simulink model "ElectricVehicleThermalManagementWithHeatPump_2026a_version"  (R2026a)
settings: Solver=VariableStepAuto  StopTime=3600  AbsTol=1e-3
PreLoadFcn:
  | init_nmpc
InitFcn:
  | init_nmpc
model workspace: external: MATLAB File ElectricVehicleThermalManagementWithHeatPumpParameters.m (data not in the file)
values from neighbouring files (symbols this model uses):
  battery_C1_LUT = [1913.6 12447 30609 ... (first row only)    [ElectricVehicleThermalManagementWithHeatPumpParameters.m]
  battery_capacity_LUT = [280.081 276.25 276.392]    [ElectricVehicleThermalManagementWithHeatPumpParameters.m]
  battery_cell_cp = 795    [ElectricVehicleThermalManagementWithHeatPumpParameters.m]
  battery_cell_mass = 2.5    [ElectricVehicleThermalManagementWithHeatPumpParameters.m]
  battery_Em_LUT = [3.4966 3.5057 3.5148 ... (first row only)    [ElectricVehicleThermalManagementWithHeatPumpParameters.m]
  battery_N_cells = 20    [ElectricVehicleThermalManagementWithHeatPumpParameters.m]
  battery_Qe_init = 0    [ElectricVehicleThermalManagementWithHeatPumpParameters.m]
  battery_R0_LUT = [0.0117 0.0085 0.009 ... (first row only)    [ElectricVehicleThermalManagementWithHeatPumpParameters.m]
  battery_R1_LUT = [0.0109 0.0029 0.0013 ... (first row only)    [ElectricVehicleThermalManagementWithHeatPumpParameters.m]
  battery_SOC_LUT = [0; 0.1; 0.25; 0.5; 0.75; 0.9; 1]    [ElectricVehicleThermalManagementWithHeatPumpParameters.m]
  battery_T_init = -5    [ElectricVehicleThermalManagementWithHeatPumpParameters.m]
  battery_temperature_LUT = [5 20 40]    [ElectricVehicleThermalManagementWithHeatPumpParameters.m]
  cabin_duct_area = 0.04    [ElectricVehicleThermalManagementWithHeatPumpParameters.m]
  cabin_T_init = -5    [ElectricVehicleThermalManagementWithHeatPumpParameters.m]
  chiller_area_primary = 0.43982297150257105    (= 0.439822971503)    [ElectricVehicleThermalManagementWithHeatPumpParameters.m]
  chiller_N_baffles = 3    [ElectricVehicleThermalManagementWithHeatPumpParameters.m]
  chiller_N_tubes = 100    [ElectricVehicleThermalManagementWithHeatPumpParameters.m]
  chiller_tube_D = 0.0035    [ElectricVehicleThermalManagementWithHeatPumpParameters.m]
  chiller_tube_L = 0.4    [ElectricVehicleThermalManagementWithHeatPumpParameters.m]
  chiller_wall_conductivity = 240    [ElectricVehicleThermalManagementWithHeatPumpParameters.m]
  chiller_wall_thickness = 0.0001    [ElectricVehicleThermalManagementWithHeatPumpParameters.m]
  cond_evap_air_area_flow = 0.3906    [ElectricVehicleThermalManagementWithHeatPumpParameters.m]
  cond_evap_air_area_primary = 1.4834999999999998    (= 1.4835)    [ElectricVehicleThermalManagementWithHeatPumpParameters.m]
  cond_evap_W = 0.015    [ElectricVehicleThermalManagementWithHeatPumpParameters.m]
  cond_evap_wall_conductivity = 240    [ElectricVehicleThermalManagementWithHeatPumpParameters.m]
  cond_evap_wall_thickness = 0.0001    [ElectricVehicleThermalManagementWithHeatPumpParameters.m]
  coolant_channel_D = 0.0092    [ElectricVehicleThermalManagementWithHeatPumpParameters.m]
  coolant_pipe_D = 0.019    [ElectricVehicleThermalManagementWithHeatPumpParameters.m]
  coolant_T_init = -5    [ElectricVehicleThermalManagementWithHeatPumpParameters.m]
  coolant_tank_area = 0.0121    [ElectricVehicleThermalManagementWithHeatPumpParameters.m]
  coolant_tank_volume = 1.25    [ElectricVehicleThermalManagementWithHeatPumpParameters.m]
  coolant_valve_D_ratio_max = 0.95    [ElectricVehicleThermalManagementWithHeatPumpParameters.m]
  coolant_valve_D_ratio_min = 0.001    [ElectricVehicleThermalManagementWithHeatPumpParameters.m]
  coolant_valve_displacement = 0.0063    [ElectricVehicleThermalManagementWithHeatPumpParameters.m]
  coolant_valve_S_max = 0.0053    [ElectricVehicleThermalManagementWithHeatPumpParameters.m]
  evaporator_air_area_flow = 0.12    [ElectricVehicleThermalManagementWithHeatPumpParameters.m]
  evaporator_air_area_primary = 0.4323    [ElectricVehicleThermalManagementWithHeatPumpParameters.m]
  evaporator_W = 0.015    [ElectricVehicleThermalManagementWithHeatPumpParameters.m]
  evaporator_wall_conductivity = 240    [ElectricVehicleThermalManagementWithHeatPumpParameters.m]
  evaporator_wall_thickness = 0.0001    [ElectricVehicleThermalManagementWithHeatPumpParameters.m]
  expansion_valve_D_ratio_max = 0.9    [ElectricVehicleThermalManagementWithHeatPumpParameters.m]
  hex_area_primary = 0.070371675440411369    (= 0.0703716754404)    [ElectricVehicleThermalManagementWithHeatPumpParameters.m]
  hex_N_tubes = 64    [ElectricVehicleThermalManagementWithHeatPumpParameters.m]
  hex_tube_D = 0.0035    [ElectricVehicleThermalManagementWithHeatPumpParameters.m]
  hex_wall_conductivity = 240    [ElectricVehicleThermalManagementWithHeatPumpParameters.m]
  hex_wall_thickness = 0.0001    [ElectricVehicleThermalManagementWithHeatPumpParameters.m]
  inner_cond_air_area_flow = 0.1953    [ElectricVehicleThermalManagementWithHeatPumpParameters.m]
  inner_cond_air_area_primary = 0.99520000000000008    (= 0.9952)    [ElectricVehicleThermalManagementWithHeatPumpParameters.m]
  inner_cond_W = 0.02    [ElectricVehicleThermalManagementWithHeatPumpParameters.m]
  inner_cond_wall_conductivity = 240    [ElectricVehicleThermalManagementWithHeatPumpParameters.m]
  inner_cond_wall_thickness = 0.0001    [ElectricVehicleThermalManagementWithHeatPumpParameters.m]
  pump_speed_max = 1000    [ElectricVehicleThermalManagementWithHeatPumpParameters.m]
  radiator_air_area_flow = 0.097499999999999989    (= 0.0975)    [ElectricVehicleThermalManagementWithHeatPumpParameters.m]
  radiator_air_area_primary = 0.43687499999999996    (= 0.436875)    [ElectricVehicleThermalManagementWithHeatPumpParameters.m]
  radiator_W = 0.015    [ElectricVehicleThermalManagementWithHeatPumpParameters.m]
  radiator_wall_conductivity = 240    [ElectricVehicleThermalManagementWithHeatPumpParameters.m]
  radiator_wall_thickness = 0.0001    [ElectricVehicleThermalManagementWithHeatPumpParameters.m]
  refrigerant_p_init = 0.25    [ElectricVehicleThermalManagementWithHeatPumpParameters.m]
  refrigerant_pipe_D = 0.01    [ElectricVehicleThermalManagementWithHeatPumpParameters.m]
  refrigerant_valve_D_ratio_max = 0.95    [ElectricVehicleThermalManagementWithHeatPumpParameters.m]
  refrigerant_valve_displacement = 0.005    [ElectricVehicleThermalManagementWithHeatPumpParameters.m]
libraries: fl_lib x227, nesl_utility x162, SimscapeFluids_lib x30, LiBatteryElements_lib x16, slpidlib x3, SignalEditorBlockLib x1
(part 11 of 13)

== system ElectricVehicleThermalManagementWithHeatPump_2026a_version/Controls/T_battery ==
  MinMax : MinMax  Function=max  Inputs=4
  T_battery : Outport
  wires:
  MinMax/1 -> T_battery/1
  [T_battery1] -> MinMax/1
  [T_battery4] -> MinMax/4
  [T_battery2] -> MinMax/2
  [T_battery3] -> MinMax/3

== system ElectricVehicleThermalManagementWithHeatPump_2026a_version/Controls/Thermal Mode ==
  note: 0 = Off
      |
      | 1 = Cold loop
      |
      | 2 = Heat pump
  T_env : Inport
  rpm_comp : Inport  Port=2
  Mode Selection : Subsystem
  Mode Transition : Subsystem
  Scope : Scope
      settings: ActiveDisplayYMinimum=0.9  ActiveDisplayYMaximum=1.1
  To Workspace : ToWorkspace  VariableName=thermal_mode  SampleTime=-1
  thermal_mode : Outport
  wires:
  T_env/1 -> Mode Selection/1(T_env)
  Mode Selection/1(setpoint) -> Scope/1, Mode Transition/1(setpoint)
  Mode Transition/1(thermal_mode) -> To Workspace/1, thermal_mode/1
  rpm_comp/1 -> Mode Transition/2(rpm_comp)

== system ElectricVehicleThermalManagementWithHeatPump_2026a_version/Controls/Valves Control ==
  thermal_mode : Inport
  T_coolant_inverter_out : Inport  Port=2
  T_coolant_battery_in : Inport  Port=3
  T_env : Inport  Port=4
  Chiller Expansion Valve : Subsystem
  Evaporator Expansion Valve : Subsystem
  Heat Pump Expansion Valve : Subsystem
  Radiator 3-Way Valve : Subsystem
  Refrigerant and Air 3-Way Valve : Subsystem
  To Workspace1 : ToWorkspace  VariableName=clntInverterTemp_out  SampleTime=-1
  To Workspace2 : ToWorkspace  VariableName=clntBatTemp_in  SampleTime=-1
  To Workspace3 : ToWorkspace  VariableName=envTemp  SampleTime=-1
  To Workspace4 : ToWorkspace  VariableName=cmdRefByPass  SampleTime=-1
  To Workspace5 : ToWorkspace  VariableName=cmdBlendAir  SampleTime=-1
  To Workspace6 : ToWorkspace  VariableName=cmdRadByPass  SampleTime=-1
  To Workspace7 : ToWorkspace  VariableName=cmdExvChill  SampleTime=-1
  To Workspace8 : ToWorkspace  VariableName=cmdExvEvap  SampleTime=-1
  To Workspace9 : ToWorkspace  VariableName=cmdExvHeatpump  SampleTime=-1
  cmd_refrig_bypass : Outport
  cmd_blend_air : Outport  Port=2
  cmd_rad_bypass : Outport  Port=3
  cmd_exv_chiller : Outport  Port=4
  cmd_exv_evap : Outport  Port=5
  cmd_exv_heatpump : Outport  Port=6
  wires:
  Refrigerant and Air 3-Way Valve/1(cmd_refrig_bypass) -> To Workspace4/1, cmd_refrig_bypass/1
  Refrigerant and Air 3-Way Valve/2(cmd_blend_air) -> To Workspace5/1, cmd_blend_air/1
  T_env/1 -> To Workspace3/1, Heat Pump Expansion Valve/2(T_env), Evaporator Expansion Valve/2(T_env)
  T_coolant_battery_in/1 -> To Workspace2/1, Chiller Expansion Valve/2(T_coolant_battery_in)
  T_coolant_inverter_out/1 -> To Workspace1/1, Radiator 3-Way Valve/2(T_coolant_inverter_out)
  thermal_mode/1 -> Radiator 3-Way Valve/1(thermal_mode), Chiller Expansion Valve/1(thermal_mode), Evaporator Expansion Valve/1(thermal_mode), Heat Pump Expansion Valve/1(thermal_mode), Refrigerant and Air 3-Way Valve/1(thermal_mode)
  Radiator 3-Way Valve/1(cmd_rad_bypass) -> To Workspace6/1, cmd_rad_bypass/1
  Chiller Expansion Valve/1(cmd_exv_chiller) -> To Workspace7/1, cmd_exv_chiller/1
  Evaporator Expansion Valve/1(cmd_exv_evap) -> To Workspace8/1, cmd_exv_evap/1
  Heat Pump Expansion Valve/1(cmd_exv_heatpump) -> To Workspace9/1, cmd_exv_heatpump/1

== system ElectricVehicleThermalManagementWithHeatPump_2026a_version/Evaporator/SR7 ==
  Flow Rate Sensor (2P) : fl_lib/Two-Phase Fluid/Sensors/Flow Rate Sensor (2P)  mass_flow_measure=true  volumetric_flow_measure=false  energy_flow_measure=true
  PS-Simulink Converter : nesl_utility/PS-Simulink Converter  PhysicalDomain=network_engine_domain  SubClassName=ps_output  LeftPortType=input  RightPortType=output  PseudoPeriodic=off  Frequencies=[]  VectorFormat=inherit  Unit=W  AffineConversion=off
  PS-Simulink Converter{1..4} (4 alike) : nesl_utility/PS-Simulink Converter  PhysicalDomain=network_engine_domain  SubClassName=ps_output  LeftPortType=input  RightPortType=output  PseudoPeriodic=off  Frequencies=[]  VectorFormat=inherit  Unit=inherit  AffineConversion=off
  "Pressure, Temperature & Internal Energy Sensor (2P)" : fl_lib/Two-Phase Fluid/Sensors/Pressure, Temperature & Internal Energy Sensor (2P)  reference=foundation.enum.MeasurementReference.absolute  pressure=true  pressure_spec=foundation.enum.PressureMeasementSpec.Absolute  temperature=false  internal_energy=false
  Thermodynamic Properties Sensor (2P) : fl_lib/Two-Phase Fluid/Sensors/Thermodynamic Properties Sensor (2P)  temperature=true  enthalpy=true  density=true  specific_volume=false  entropy=true
  To Workspace : ToWorkspace  VariableName=refEvapTemp_in  SampleTime=-1
  To Workspace1 : ToWorkspace  VariableName=refEvapH_in  SampleTime=-1
  To Workspace2 : ToWorkspace  VariableName=refEvapRho_in  SampleTime=-1
  To Workspace3 : ToWorkspace  VariableName=refEvapPres_in  SampleTime=-1
  A : PMIOPort  Side=Left
  B : PMIOPort  Port=2  Side=Right
  tag scope: Phi_evap_in=global
  wires:
  PS-Simulink Converter/1 -> [Phi_evap_in]
  PS-Simulink Converter1/1 -> To Workspace/1
  PS-Simulink Converter2/1 -> To Workspace1/1
  PS-Simulink Converter3/1 -> To Workspace2/1
  PS-Simulink Converter4/1 -> To Workspace3/1
  connections:
  PS-Simulink Converter/LConn1 -- Flow Rate Sensor (2P)/RConn3
  B/RConn1 -- Flow Rate Sensor (2P)/RConn1
  Thermodynamic Properties Sensor (2P)/LConn1 -- A/RConn1 -- "Pressure, Temperature & Internal Energy Sensor (2P)"/LConn1 -- Flow Rate Sensor (2P)/LConn1
  PS-Simulink Converter1/LConn1 -- Thermodynamic Properties Sensor (2P)/RConn1
  PS-Simulink Converter2/LConn1 -- Thermodynamic Properties Sensor (2P)/RConn2
  PS-Simulink Converter3/LConn1 -- Thermodynamic Properties Sensor (2P)/RConn3
  PS-Simulink Converter4/LConn1 -- "Pressure, Temperature & Internal Energy Sensor (2P)"/RConn1

== system ElectricVehicleThermalManagementWithHeatPump_2026a_version/Evaporator/SR8 ==
  Flow Rate Sensor (2P) : fl_lib/Two-Phase Fluid/Sensors/Flow Rate Sensor (2P)  mass_flow_measure=true  volumetric_flow_measure=false  energy_flow_measure=true
  PS-Simulink Converter : nesl_utility/PS-Simulink Converter  PhysicalDomain=network_engine_domain  SubClassName=ps_output  LeftPortType=input  RightPortType=output  PseudoPeriodic=off  Frequencies=[]  VectorFormat=inherit  Unit=W  AffineConversion=off
  PS-Simulink Converter1 : nesl_utility/PS-Simulink Converter  PhysicalDomain=network_engine_domain  SubClassName=ps_output  LeftPortType=input  RightPortType=output  PseudoPeriodic=off  Frequencies=[]  VectorFormat=inherit  Unit=MPa  AffineConversion=off
  PS-Simulink Converter2 : nesl_utility/PS-Simulink Converter  PhysicalDomain=network_engine_domain  SubClassName=ps_output  LeftPortType=input  RightPortType=output  PseudoPeriodic=off  Frequencies=[]  VectorFormat=inherit  Unit=inherit  AffineConversion=off
  PS-Simulink Converter3 : nesl_utility/PS-Simulink Converter  PhysicalDomain=network_engine_domain  SubClassName=ps_output  LeftPortType=input  RightPortType=output  PseudoPeriodic=off  Frequencies=[]  VectorFormat=inherit  Unit=inherit  AffineConversion=off
  PS-Simulink Converter4 : nesl_utility/PS-Simulink Converter  PhysicalDomain=network_engine_domain  SubClassName=ps_output  LeftPortType=input  RightPortType=output  PseudoPeriodic=off  Frequencies=[]  VectorFormat=inherit  Unit=inherit  AffineConversion=off
  "Pressure, Temperature & Internal Energy Sensor (2P)" : fl_lib/Two-Phase Fluid/Sensors/Pressure, Temperature & Internal Energy Sensor (2P)  reference=foundation.enum.MeasurementReference.absolute  pressure=true  pressure_spec=foundation.enum.PressureMeasementSpec.Absolute  temperature=false  internal_energy=false
  Thermodynamic Properties Sensor (2P) : fl_lib/Two-Phase Fluid/Sensors/Thermodynamic Properties Sensor (2P)  temperature=true  enthalpy=true  density=true  specific_volume=false  entropy=true
  To Workspace : ToWorkspace  VariableName=refEvapPress_out  SampleTime=-1
  To Workspace1 : ToWorkspace  VariableName=refEvapTemp_out  SampleTime=-1
  To Workspace2 : ToWorkspace  VariableName=refEvapH_out  SampleTime=-1
  To Workspace3 : ToWorkspace  VariableName=refEvapRho_out  SampleTime=-1
  A : PMIOPort  Side=Left
  B : PMIOPort  Port=2  Side=Right
  tag scope: Phi_evap_out=global, p_evap_out=global
  wires:
  PS-Simulink Converter/1 -> [Phi_evap_out]
  PS-Simulink Converter1/1 -> To Workspace/1, [p_evap_out]
  PS-Simulink Converter2/1 -> To Workspace1/1
  PS-Simulink Converter3/1 -> To Workspace2/1
  PS-Simulink Converter4/1 -> To Workspace3/1
  connections:
  PS-Simulink Converter/LConn1 -- Flow Rate Sensor (2P)/RConn3
  B/RConn1 -- Flow Rate Sensor (2P)/RConn1
  Thermodynamic Properties Sensor (2P)/LConn1 -- A/RConn1 -- "Pressure, Temperature & Internal Energy Sensor (2P)"/LConn1 -- Flow Rate Sensor (2P)/LConn1
  PS-Simulink Converter1/LConn1 -- "Pressure, Temperature & Internal Energy Sensor (2P)"/RConn1
  PS-Simulink Converter2/LConn1 -- Thermodynamic Properties Sensor (2P)/RConn1
  PS-Simulink Converter3/LConn1 -- Thermodynamic Properties Sensor (2P)/RConn2
  PS-Simulink Converter4/LConn1 -- Thermodynamic Properties Sensor (2P)/RConn3

== system ElectricVehicleThermalManagementWithHeatPump_2026a_version/Heat Exchanger/SR5 ==
  Flow Rate Sensor (2P) : fl_lib/Two-Phase Fluid/Sensors/Flow Rate Sensor (2P)  mass_flow_measure=true  volumetric_flow_measure=false  energy_flow_measure=true
  PS-Simulink Converter : nesl_utility/PS-Simulink Converter  PhysicalDomain=network_engine_domain  SubClassName=ps_output  LeftPortType=input  RightPortType=output  PseudoPeriodic=off  Frequencies=[]  VectorFormat=inherit  Unit=W  AffineConversion=off
  PS-Simulink Converter1 : nesl_utility/PS-Simulink Converter  PhysicalDomain=network_engine_domain  SubClassName=ps_output  LeftPortType=input  RightPortType=output  PseudoPeriodic=off  Frequencies=[]  VectorFormat=inherit  Unit=inherit  AffineConversion=off
  PS-Simulink Converter2 : nesl_utility/PS-Simulink Converter  PhysicalDomain=network_engine_domain  SubClassName=ps_output  LeftPortType=input  RightPortType=output  PseudoPeriodic=off  Frequencies=[]  VectorFormat=inherit  Unit=inherit  AffineConversion=off
  PS-Simulink Converter3 : nesl_utility/PS-Simulink Converter  PhysicalDomain=network_engine_domain  SubClassName=ps_output  LeftPortType=input  RightPortType=output  PseudoPeriodic=off  Frequencies=[]  VectorFormat=inherit  Unit=inherit  AffineConversion=off
  "Pressure, Temperature & Internal Energy Sensor (2P)" : fl_lib/Two-Phase Fluid/Sensors/Pressure, Temperature & Internal Energy Sensor (2P)  reference=foundation.enum.MeasurementReference.absolute  pressure=true  pressure_spec=foundation.enum.PressureMeasementSpec.Absolute  temperature=false  internal_energy=false
  Scope : Scope
      settings: DataLoggingVariableName=ScopeData4
  Scope1 : Scope
      settings: ActiveDisplayYMinimum=256.57304  ActiveDisplayYMaximum=268.20044  DataLoggingVariableName=ScopeData5
  Scope2 : Scope
      settings: DataLoggingVariableName=ScopeData6
  Thermodynamic Properties Sensor (2P) : fl_lib/Two-Phase Fluid/Sensors/Thermodynamic Properties Sensor (2P)  temperature=true  enthalpy=true  density=true  specific_volume=false  entropy=true
  To Workspace : ToWorkspace  VariableName=heatExchangerRefPress_inPa  SampleTime=-1
  To Workspace1 : ToWorkspace  VariableName=heatExchangerRefTemp_inK  SampleTime=-1
  To Workspace2 : ToWorkspace  VariableName=heatExchangerRefEnthaply_in  SampleTime=-1
  A : PMIOPort  Side=Left
  B : PMIOPort  Port=2  Side=Right
  tag scope: Phi_hex_in=global
  wires:
  PS-Simulink Converter/1 -> [Phi_hex_in]
  PS-Simulink Converter2/1 -> Scope/1, To Workspace/1
  PS-Simulink Converter1/1 -> Scope1/1, To Workspace1/1
  PS-Simulink Converter3/1 -> Scope2/1, To Workspace2/1
  connections:
  PS-Simulink Converter/LConn1 -- Flow Rate Sensor (2P)/RConn3
  B/RConn1 -- Flow Rate Sensor (2P)/RConn1
  Thermodynamic Properties Sensor (2P)/LConn1 -- A/RConn1 -- "Pressure, Temperature & Internal Energy Sensor (2P)"/LConn1 -- Flow Rate Sensor (2P)/LConn1
  PS-Simulink Converter1/LConn1 -- Thermodynamic Properties Sensor (2P)/RConn1
  PS-Simulink Converter2/LConn1 -- "Pressure, Temperature & Internal Energy Sensor (2P)"/RConn1
  Thermodynamic Properties Sensor (2P)/RConn2 -- PS-Simulink Converter3/LConn1

== system ElectricVehicleThermalManagementWithHeatPump_2026a_version/Heat Exchanger/SR6 ==
  Flow Rate Sensor (2P) : fl_lib/Two-Phase Fluid/Sensors/Flow Rate Sensor (2P)  mass_flow_measure=true  volumetric_flow_measure=false  energy_flow_measure=true
  PS-Simulink Converter : nesl_utility/PS-Simulink Converter  PhysicalDomain=network_engine_domain  SubClassName=ps_output  LeftPortType=input  RightPortType=output  PseudoPeriodic=off  Frequencies=[]  VectorFormat=inherit  Unit=W  AffineConversion=off
  PS-Simulink Converter1 : nesl_utility/PS-Simulink Converter  PhysicalDomain=network_engine_domain  SubClassName=ps_output  LeftPortType=input  RightPortType=output  PseudoPeriodic=off  Frequencies=[]  VectorFormat=inherit  Unit=inherit  AffineConversion=off
  PS-Simulink Converter2 : nesl_utility/PS-Simulink Converter  PhysicalDomain=network_engine_domain  SubClassName=ps_output  LeftPortType=input  RightPortType=output  PseudoPeriodic=off  Frequencies=[]  VectorFormat=inherit  Unit=inherit  AffineConversion=off
  PS-Simulink Converter3 : nesl_utility/PS-Simulink Converter  PhysicalDomain=network_engine_domain  SubClassName=ps_output  LeftPortType=input  RightPortType=output  PseudoPeriodic=off  Frequencies=[]  VectorFormat=inherit  Unit=inherit  AffineConversion=off
  "Pressure, Temperature & Internal Energy Sensor (2P)" : fl_lib/Two-Phase Fluid/Sensors/Pressure, Temperature & Internal Energy Sensor (2P)  reference=foundation.enum.MeasurementReference.absolute  pressure=true  pressure_spec=foundation.enum.PressureMeasementSpec.Absolute  temperature=false  internal_energy=false
  Scope : Scope
      settings: DataLoggingVariableName=ScopeData7
  Scope1 : Scope
      settings: ActiveDisplayYMinimum=256.25115  ActiveDisplayYMaximum=271.0073  DataLoggingVariableName=ScopeData8
  Scope2 : Scope
      settings: DataLoggingVariableName=ScopeData9
  Thermodynamic Properties Sensor (2P) : fl_lib/Two-Phase Fluid/Sensors/Thermodynamic Properties Sensor (2P)  temperature=true  enthalpy=true  density=true  specific_volume=false  entropy=true
  To Workspace : ToWorkspace  VariableName=heatExchangerRefPress_outPa  SampleTime=-1
  To Workspace1 : ToWorkspace  VariableName=heatExchangerRefTemp_outK  SampleTime=-1
  To Workspace2 : ToWorkspace  VariableName=heatExchangerRefEnthaply_out  SampleTime=-1
  A : PMIOPort  Side=Left
  B : PMIOPort  Port=2  Side=Right
  tag scope: Phi_hex_out=global
  wires:
  PS-Simulink Converter/1 -> [Phi_hex_out]
  PS-Simulink Converter1/1 -> Scope/1, To Workspace/1
  PS-Simulink Converter2/1 -> Scope1/1, To Workspace1/1
  PS-Simulink Converter3/1 -> Scope2/1, To Workspace2/1
  connections:
  PS-Simulink Converter/LConn1 -- Flow Rate Sensor (2P)/RConn3
  B/RConn1 -- Flow Rate Sensor (2P)/RConn1
  Thermodynamic Properties Sensor (2P)/LConn1 -- A/RConn1 -- "Pressure, Temperature & Internal Energy Sensor (2P)"/LConn1 -- Flow Rate Sensor (2P)/LConn1
  PS-Simulink Converter1/LConn1 -- "Pressure, Temperature & Internal Energy Sensor (2P)"/RConn1
  PS-Simulink Converter2/LConn1 -- Thermodynamic Properties Sensor (2P)/RConn1
  PS-Simulink Converter3/LConn1 -- Thermodynamic Properties Sensor (2P)/RConn2

== system ElectricVehicleThermalManagementWithHeatPump_2026a_version/Inner Condenser/SR1 ==
  Flow Rate Sensor (2P) : fl_lib/Two-Phase Fluid/Sensors/Flow Rate Sensor (2P)  mass_flow_measure=true  volumetric_flow_measure=false  energy_flow_measure=true
  PS-Simulink Converter : nesl_utility/PS-Simulink Converter  PhysicalDomain=network_engine_domain  SubClassName=ps_output  LeftPortType=input  RightPortType=output  PseudoPeriodic=off  Frequencies=[]  VectorFormat=inherit  Unit=W  AffineConversion=off
  PS-Simulink Converter{1..4} (4 alike) : nesl_utility/PS-Simulink Converter  PhysicalDomain=network_engine_domain  SubClassName=ps_output  LeftPortType=input  RightPortType=output  PseudoPeriodic=off  Frequencies=[]  VectorFormat=inherit  Unit=inherit  AffineConversion=off
  "Pressure, Temperature & Internal Energy Sensor (2P)" : fl_lib/Two-Phase Fluid/Sensors/Pressure, Temperature & Internal Energy Sensor (2P)  reference=foundation.enum.MeasurementReference.absolute  pressure=true  pressure_spec=foundation.enum.PressureMeasementSpec.Absolute  temperature=false  internal_energy=false
  Scope{,1..3} (4 alike) : Scope
      Scope settings: DataLoggingVariableName=ScopeData13
      Scope1 settings: ActiveDisplayYMinimum=-0.00405  ActiveDisplayYMaximum=0.03648  DataLoggingVariableName=ScopeData14
      Scope2 settings: ActiveDisplayYMinimum=241.8446  ActiveDisplayYMaximum=454.07101  DataLoggingVariableName=ScopeData15
      Scope3 settings: DataLoggingVariableName=ScopeData16
  Thermodynamic Properties Sensor (2P) : fl_lib/Two-Phase Fluid/Sensors/Thermodynamic Properties Sensor (2P)  temperature=true  enthalpy=true  density=true  specific_volume=false  entropy=true
  To Workspace : ToWorkspace  VariableName=innerCondRefPress_inMPa  SampleTime=-1
  To Workspace1 : ToWorkspace  VariableName=RefMassFlowRate  SampleTime=-1
  To Workspace2 : ToWorkspace  VariableName=innerCondRefTemp_inK  SampleTime=-1
  To Workspace3 : ToWorkspace  VariableName=innerCondRefEnthaply_in  SampleTime=-1
  A : PMIOPort  Side=Left
  B : PMIOPort  Port=2  Side=Right
  tag scope: Phi_inner_cond_in=global
  wires:
  PS-Simulink Converter/1 -> [Phi_inner_cond_in]
  PS-Simulink Converter1/1 -> Scope/1, To Workspace/1
  PS-Simulink Converter2/1 -> Scope1/1, To Workspace1/1
  PS-Simulink Converter3/1 -> Scope2/1, To Workspace2/1
  PS-Simulink Converter4/1 -> Scope3/1, To Workspace3/1
  connections:
  PS-Simulink Converter/LConn1 -- Flow Rate Sensor (2P)/RConn3
  B/RConn1 -- Flow Rate Sensor (2P)/RConn1
  Thermodynamic Properties Sensor (2P)/LConn1 -- A/RConn1 -- "Pressure, Temperature & Internal Energy Sensor (2P)"/LConn1 -- Flow Rate Sensor (2P)/LConn1
  PS-Simulink Converter1/LConn1 -- "Pressure, Temperature & Internal Energy Sensor (2P)"/RConn1
  PS-Simulink Converter2/LConn1 -- Flow Rate Sensor (2P)/RConn2
  PS-Simulink Converter3/LConn1 -- Thermodynamic Properties Sensor (2P)/RConn1
  PS-Simulink Converter4/LConn1 -- Thermodynamic Properties Sensor (2P)/RConn2

== system ElectricVehicleThermalManagementWithHeatPump_2026a_version/Inner Condenser/SR2 ==
  Flow Rate Sensor (2P) : fl_lib/Two-Phase Fluid/Sensors/Flow Rate Sensor (2P)  mass_flow_measure=true  volumetric_flow_measure=false  energy_flow_measure=true
  PS-Simulink Converter : nesl_utility/PS-Simulink Converter  PhysicalDomain=network_engine_domain  SubClassName=ps_output  LeftPortType=input  RightPortType=output  PseudoPeriodic=off  Frequencies=[]  VectorFormat=inherit  Unit=W  AffineConversion=off
  PS-Simulink Converter1 : nesl_utility/PS-Simulink Converter  PhysicalDomain=network_engine_domain  SubClassName=ps_output  LeftPortType=input  RightPortType=output  PseudoPeriodic=off  Frequencies=[]  VectorFormat=inherit  Unit=MPa  AffineConversion=off
  PS-Simulink Converter2 : nesl_utility/PS-Simulink Converter  PhysicalDomain=network_engine_domain  SubClassName=ps_output  LeftPortType=input  RightPortType=output  PseudoPeriodic=off  Frequencies=[]  VectorFormat=inherit  Unit=inherit  AffineConversion=off
  PS-Simulink Converter3 : nesl_utility/PS-Simulink Converter  PhysicalDomain=network_engine_domain  SubClassName=ps_output  LeftPortType=input  RightPortType=output  PseudoPeriodic=off  Frequencies=[]  VectorFormat=inherit  Unit=inherit  AffineConversion=off
  "Pressure, Temperature & Internal Energy Sensor (2P)" : fl_lib/Two-Phase Fluid/Sensors/Pressure, Temperature & Internal Energy Sensor (2P)  reference=foundation.enum.MeasurementReference.absolute  pressure=true  pressure_spec=foundation.enum.PressureMeasementSpec.Absolute  temperature=false  internal_energy=false
  Thermodynamic Properties Sensor (2P) : fl_lib/Two-Phase Fluid/Sensors/Thermodynamic Properties Sensor (2P)  temperature=true  enthalpy=true  density=true  specific_volume=false  entropy=true
  To Workspace : ToWorkspace  VariableName=innerCondRefPress_outMpa  SampleTime=-1
  To Workspace1 : ToWorkspace  VariableName=innerCondRefTemp_outK  SampleTime=-1
  To Workspace2 : ToWorkspace  VariableName=innerCondRefEnthaply_out  SampleTime=-1
  A : PMIOPort  Side=Left
  B : PMIOPort  Port=2  Side=Right
  tag scope: Phi_inner_cond_out=global, p_inner_cond_out=global
  wires:
  PS-Simulink Converter/1 -> [Phi_inner_cond_out]
  PS-Simulink Converter1/1 -> To Workspace/1, [p_inner_cond_out]
  PS-Simulink Converter2/1 -> To Workspace1/1
  PS-Simulink Converter3/1 -> To Workspace2/1
  connections:
  PS-Simulink Converter/LConn1 -- Flow Rate Sensor (2P)/RConn3
  B/RConn1 -- Flow Rate Sensor (2P)/RConn1
  Thermodynamic Properties Sensor (2P)/LConn1 -- A/RConn1 -- "Pressure, Temperature & Internal Energy Sensor (2P)"/LConn1 -- Flow Rate Sensor (2P)/LConn1
  PS-Simulink Converter1/LConn1 -- "Pressure, Temperature & Internal Energy Sensor (2P)"/RConn1
  PS-Simulink Converter2/LConn1 -- Thermodynamic Properties Sensor (2P)/RConn1
  PS-Simulink Converter3/LConn1 -- Thermodynamic Properties Sensor (2P)/RConn2

== system ElectricVehicleThermalManagementWithHeatPump_2026a_version/Inverter/SC7 ==
  Flow Rate Sensor (TL) : fl_lib/Thermal Liquid/Sensors/Flow Rate Sensor (TL)  mass_flow_measure=true  volumetric_flow_measure=false  energy_flow_measure=true
  PS-Simulink Converter1 : nesl_utility/PS-Simulink Converter  PhysicalDomain=network_engine_domain  SubClassName=ps_output  LeftPortType=input  RightPortType=output  PseudoPeriodic=off  Frequencies=[]  VectorFormat=inherit  Unit=degC  AffineConversion=on
  Pressure & Temperature Sensor (TL) : fl_lib/Thermal Liquid/Sensors/Pressure & Temperature Sensor (TL)  reference=foundation.enum.MeasurementReference.absolute  pressure=true  pressure_spec=foundation.enum.PressureMeasementSpec.Absolute  temperature=true
  A : PMIOPort  Side=Left
  B : PMIOPort  Port=2  Side=Right
  tag scope: T_coolant_inverter_out=global
  wires:
  PS-Simulink Converter1/1 -> [T_coolant_inverter_out]
  connections:
  B/RConn1 -- Flow Rate Sensor (TL)/RConn1
  Flow Rate Sensor (TL)/LConn1 -- Pressure & Temperature Sensor (TL)/LConn1 -- A/RConn1
  PS-Simulink Converter1/LConn1 -- Pressure & Temperature Sensor (TL)/RConn2

== system ElectricVehicleThermalManagementWithHeatPump_2026a_version/Motor/SC5 ==
  Flow Rate Sensor (TL) : fl_lib/Thermal Liquid/Sensors/Flow Rate Sensor (TL)  mass_flow_measure=true  volumetric_flow_measure=false  energy_flow_measure=true
  PS-Simulink Converter : nesl_utility/PS-Simulink Converter  PhysicalDomain=network_engine_domain  SubClassName=ps_output  LeftPortType=input  RightPortType=output  PseudoPeriodic=off  Frequencies=[]  VectorFormat=inherit  Unit=W  AffineConversion=off
  Pressure & Temperature Sensor (TL) : fl_lib/Thermal Liquid/Sensors/Pressure & Temperature Sensor (TL)  reference=foundation.enum.MeasurementReference.absolute  pressure=true  pressure_spec=foundation.enum.PressureMeasementSpec.Absolute  temperature=true
  A : PMIOPort  Side=Left
  B : PMIOPort  Port=2  Side=Right
  tag scope: Phi_motor_in=global
  wires:
  PS-Simulink Converter/1 -> [Phi_motor_in]
  connections:
  B/RConn1 -- Flow Rate Sensor (TL)/RConn1
  Flow Rate Sensor (TL)/LConn1 -- Pressure & Temperature Sensor (TL)/LConn1 -- A/RConn1
  PS-Simulink Converter/LConn1 -- Flow Rate Sensor (TL)/RConn3

== system ElectricVehicleThermalManagementWithHeatPump_2026a_version/Motor/SC6 ==
  Flow Rate Sensor (TL) : fl_lib/Thermal Liquid/Sensors/Flow Rate Sensor (TL)  mass_flow_measure=true  volumetric_flow_measure=false  energy_flow_measure=true
  PS-Simulink Converter : nesl_utility/PS-Simulink Converter  PhysicalDomain=network_engine_domain  SubClassName=ps_output  LeftPortType=input  RightPortType=output  PseudoPeriodic=off  Frequencies=[]  VectorFormat=inherit  Unit=W  AffineConversion=off
  Pressure & Temperature Sensor (TL) : fl_lib/Thermal Liquid/Sensors/Pressure & Temperature Sensor (TL)  reference=foundation.enum.MeasurementReference.absolute  pressure=true  pressure_spec=foundation.enum.PressureMeasementSpec.Absolute  temperature=true
  A : PMIOPort  Side=Left
  B : PMIOPort  Port=2  Side=Right
  tag scope: Phi_motor_out=global
  wires:
  PS-Simulink Converter/1 -> [Phi_motor_out]
  connections:
  B/RConn1 -- Flow Rate Sensor (TL)/RConn1
  Flow Rate Sensor (TL)/LConn1 -- Pressure & Temperature Sensor (TL)/LConn1 -- A/RConn1
  PS-Simulink Converter/LConn1 -- Flow Rate Sensor (TL)/RConn3

== system ElectricVehicleThermalManagementWithHeatPump_2026a_version/Motor Pump/Heat Transfer ==
  Convective Heat Transfer : fl_lib/Thermal/Thermal Elements/Convective Heat Transfer  thermal_type=foundation.enum.constant_variable.constant  area=3 * coolant_tank_area m^2  heat_tr_coeff=20 W/(m^2 * K)  min_heat_tr_coeff=1e-3 W/(K*m^2)  T_specify=off  T_priority=None  T=0 K  T_nominal_specify=off  T_nominal_value=1  T_nominal_unit=K  Q_specify=off  Q_priority=None  Q=0 W  Q_nominal_specify=off  Q_nominal_value=1  Q_nominal_unit=W
  Convective Heat Transfer1 : fl_lib/Thermal/Thermal Elements/Convective Heat Transfer  thermal_type=foundation.enum.constant_variable.constant  area=3 * coolant_tank_area m^2  heat_tr_coeff=20 W/(m^2 * K)  min_heat_tr_coeff=1e-3 W/(K*m^2)  T_specify=off  T_priority=None  T=0 K  T_nominal_specify=off  T_nominal_value=1  T_nominal_unit=K  Q_specify=off  Q_priority=None  Q=0 W  Q_nominal_specify=off  Q_nominal_value=1  Q_nominal_unit=W
  Environment Temperature : fl_lib/Thermal/Thermal Sources/Controlled Temperature Source
  Simulink-PS Converter : nesl_utility/Simulink-PS Converter  PhysicalDomain=network_engine_domain  SubClassName=ps_input  LeftPortType=input  RightPortType=output  PseudoPeriodic=off  Frequencies=[]  NoiseDistribution=none  NoiseParameters=[]  Unit=degC  AffineConversion=on  FilteringAndDerivatives=provide  SimscapeFilterOrder=1  InputFilterTimeConstant=0.001  UdotUserProvided=0
  Thermal Reference : fl_lib/Thermal/Thermal Elements/Thermal Reference
  A : PMIOPort  Side=Right
  B : PMIOPort  Port=2  Side=Right
  wires:
  [T_env] -> Simulink-PS Converter/1
  connections:
  Simulink-PS Converter/RConn1 -- Environment Temperature/RConn1
  Thermal Reference/LConn1 -- Environment Temperature/RConn2
  Convective Heat Transfer/RConn1 -- Environment Temperature/LConn1 -- Convective Heat Transfer1/RConn1
  B/RConn1 -- Convective Heat Transfer1/LConn1
  A/RConn1 -- Convective Heat Transfer/LConn1

== system ElectricVehicleThermalManagementWithHeatPump_2026a_version/Radiator/SC1 ==
  Flow Rate Sensor (TL) : fl_lib/Thermal Liquid/Sensors/Flow Rate Sensor (TL)  mass_flow_measure=true  volumetric_flow_measure=false  energy_flow_measure=true
  PS-Simulink Converter : nesl_utility/PS-Simulink Converter  PhysicalDomain=network_engine_domain  SubClassName=ps_output  LeftPortType=input  RightPortType=output  PseudoPeriodic=off  Frequencies=[]  VectorFormat=inherit  Unit=W  AffineConversion=off
  PS-Simulink Converter1 : nesl_utility/PS-Simulink Converter  PhysicalDomain=network_engine_domain  SubClassName=ps_output  LeftPortType=input  RightPortType=output  PseudoPeriodic=off  Frequencies=[]  VectorFormat=inherit  Unit=inherit  AffineConversion=off
  Pressure & Temperature Sensor (TL) : fl_lib/Thermal Liquid/Sensors/Pressure & Temperature Sensor (TL)  reference=foundation.enum.MeasurementReference.absolute  pressure=true  pressure_spec=foundation.enum.PressureMeasementSpec.Absolute  temperature=true
  To Workspace : ToWorkspace  VariableName=clntRadTemp_in  SampleTime=-1
  A : PMIOPort  Side=Left
  B : PMIOPort  Port=2  Side=Right
  tag scope: Phi_rad_in=global
  wires:
  PS-Simulink Converter/1 -> [Phi_rad_in]
  PS-Simulink Converter1/1 -> To Workspace/1
  connections:
  PS-Simulink Converter/LConn1 -- Flow Rate Sensor (TL)/RConn3
  A/RConn1 -- Pressure & Temperature Sensor (TL)/LConn1 -- Flow Rate Sensor (TL)/LConn1
  B/RConn1 -- Flow Rate Sensor (TL)/RConn1
  PS-Simulink Converter1/LConn1 -- Pressure & Temperature Sensor (TL)/RConn2

== system ElectricVehicleThermalManagementWithHeatPump_2026a_version/Radiator/SC2 ==
  Flow Rate Sensor (TL) : fl_lib/Thermal Liquid/Sensors/Flow Rate Sensor (TL)  mass_flow_measure=true  volumetric_flow_measure=false  energy_flow_measure=true
  PS-Simulink Converter : nesl_utility/PS-Simulink Converter  PhysicalDomain=network_engine_domain  SubClassName=ps_output  LeftPortType=input  RightPortType=output  PseudoPeriodic=off  Frequencies=[]  VectorFormat=inherit  Unit=W  AffineConversion=off
  PS-Simulink Converter1 : nesl_utility/PS-Simulink Converter  PhysicalDomain=network_engine_domain  SubClassName=ps_output  LeftPortType=input  RightPortType=output  PseudoPeriodic=off  Frequencies=[]  VectorFormat=inherit  Unit=kg/s  AffineConversion=off
  PS-Simulink Converter2 : nesl_utility/PS-Simulink Converter  PhysicalDomain=network_engine_domain  SubClassName=ps_output  LeftPortType=input  RightPortType=output  PseudoPeriodic=off  Frequencies=[]  VectorFormat=inherit  Unit=inherit  AffineConversion=off
  Pressure & Temperature Sensor (TL) : fl_lib/Thermal Liquid/Sensors/Pressure & Temperature Sensor (TL)  reference=foundation.enum.MeasurementReference.absolute  pressure=true  pressure_spec=foundation.enum.PressureMeasementSpec.Absolute  temperature=true
  Scope : Scope
      settings: ActiveDisplayYMinimum=-0.01333  ActiveDisplayYMaximum=0.11994  DataLoggingVariableName=ScopeData4
  To Workspace : ToWorkspace  VariableName=clntRadTemp_out  SampleTime=-1
  A : PMIOPort  Side=Left
  B : PMIOPort  Port=2  Side=Right
  tag scope: Phi_rad_out=global
  wires:
  PS-Simulink Converter/1 -> [Phi_rad_out]
  PS-Simulink Converter1/1 -> Scope/1
  PS-Simulink Converter2/1 -> To Workspace/1
  connections:
  PS-Simulink Converter/LConn1 -- Flow Rate Sensor (TL)/RConn3
  A/RConn1 -- Pressure & Temperature Sensor (TL)/LConn1 -- Flow Rate Sensor (TL)/LConn1
  B/RConn1 -- Flow Rate Sensor (TL)/RConn1
  PS-Simulink Converter1/LConn1 -- Flow Rate Sensor (TL)/RConn2
  PS-Simulink Converter2/LConn1 -- Pressure & Temperature Sensor (TL)/RConn2

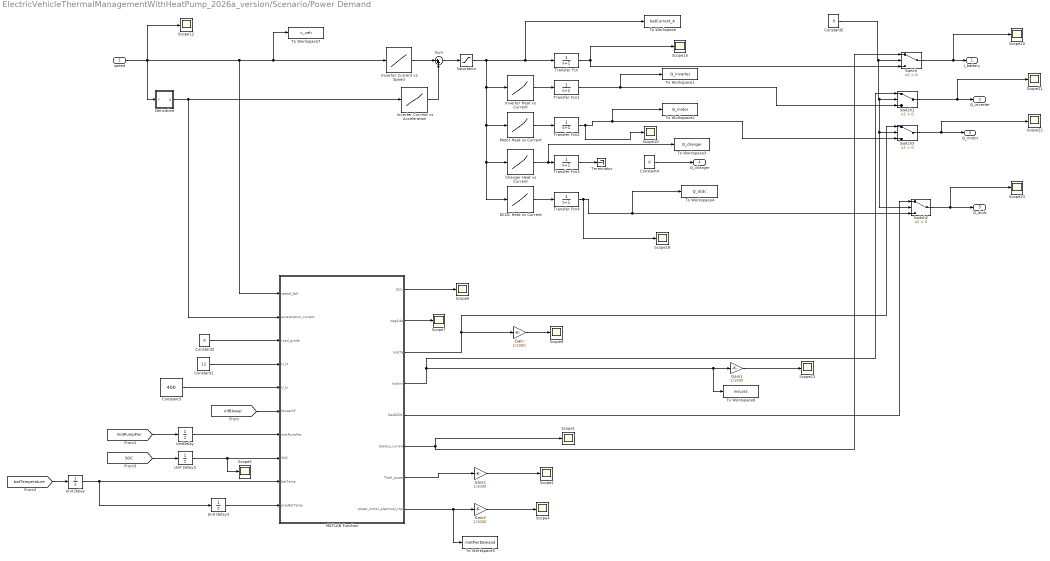
== system ElectricVehicleThermalManagementWithHeatPump_2026a_version/Scenario/Power Demand ==
  speed : Inport
  Charger Heat vs Current : Lookup_n-D  NumberOfTableDimensions=1  BreakpointsForDimension1=[-100 0 25 50 300]  IndexSearchMethod=Linear search  BeginIndexSearchUsingPreviousIndexResult=on  Table=[250 0 40 70 400]  InternalRulePriority=Speed  RndMeth=Simplest
  Constant1 : Constant  Value=12
  Constant2 : Constant  Value=0
  Constant3 : Constant  Value=400
  Constant4 : Constant  Value=0
  Constant5 : Constant  Value=0
  DCDC Heat vs Current : Lookup_n-D  NumberOfTableDimensions=1  BreakpointsForDimension1=[-100 0 25 50 300]  IndexSearchMethod=Linear search  BeginIndexSearchUsingPreviousIndexResult=on  Table=[250 0 40 70 400]  InternalRulePriority=Speed  RndMeth=Simplest
  Derivative : Subsystem  mask(1-st Order Filter Derivative){tau=1}
      mask prompts: tau "Filter time constant [s]"
  Gain{,1..3} (4 alike) : Gain  Gain=1/1000
  Inverter Current vs Acceleration : Lookup_n-D  NumberOfTableDimensions=1  BreakpointsForDimension1=[-10 -8 -5 0 5 8 10]  IndexSearchMethod=Linear search  BeginIndexSearchUsingPreviousIndexResult=on  Table=[200 150 100 0 100 150 200]*0.6  InternalRulePriority=Speed  RndMeth=Simplest
  Inverter Current vs Speed : Lookup_n-D  NumberOfTableDimensions=1  BreakpointsForDimension1=[0 60 80 100 120 140 160 180 200]  IndexSearchMethod=Linear search  BeginIndexSearchUsingPreviousIndexResult=on  Table=[0 10 18 27 45 65 100 120 160]  InternalRulePriority=Speed  RndMeth=Simplest
  Inverter Heat vs Current : Lookup_n-D  NumberOfTableDimensions=1  BreakpointsForDimension1=[-100 0 25 50 300]  IndexSearchMethod=Linear search  BeginIndexSearchUsingPreviousIndexResult=on  Table=[250 0 40 70 400]  InternalRulePriority=Speed  RndMeth=Simplest
  MATLAB Function : MATLAB Function  TreatAsAtomicUnit=on
  Motor Heat vs Current : Lookup_n-D  NumberOfTableDimensions=1  BreakpointsForDimension1=[-150 -70 -26 0 25 50 100 300 600]  IndexSearchMethod=Linear search  BeginIndexSearchUsingPreviousIndexResult=on  Table=[3500 2650 2100 0 400 550 4800 4800 4800]  InternalRulePriority=Speed  RndMeth=Simplest
  Saturation : Saturate  UpperLimit=200  LowerLimit=-inf  ZeroCross=off
  Scope{1..2,4..8,10,12..13,15..16,20..23} (16 alike) : Scope
      Scope1 settings: ActiveDisplayYMinimum=-304.69797  ActiveDisplayYMaximum=313.76479
      Scope10 settings: ActiveDisplayYMinimum=-961.00961  ActiveDisplayYMaximum=511.434  DataLoggingVariableName=ScopeData3
      Scope12 settings: ActiveDisplayYMinimum=-16.25  ActiveDisplayYMaximum=146.25  DataLoggingVariableName=ScopeData5
      Scope13 settings: ActiveDisplayYMinimum=-0.53095  ActiveDisplayYMaximum=4.77853  DataLoggingVariableName=ScopeData6
      Scope15 settings: ActiveDisplayYMinimum=-21.87365  ActiveDisplayYMaximum=196.86281
      Scope16 settings: DataLoggingVariableName=ScopeData9
      Scope2 settings: ActiveDisplayYMinimum=-153.73707  ActiveDisplayYMaximum=160.788  DataLoggingVariableName=ScopeData2
      Scope20 settings: ActiveDisplayYMinimum=-304.69797  ActiveDisplayYMaximum=313.76479  DataLoggingVariableName=ScopeData4
      Scope21 settings: DataLoggingVariableName=ScopeData5
      Scope22 settings: DataLoggingVariableName=ScopeData6
      Scope23 settings: DataLoggingVariableName=ScopeData7
      Scope4 settings: ActiveDisplayYMinimum=-153.48116  ActiveDisplayYMaximum=158.4825
      Scope5 settings: ActiveDisplayYMinimum=-153.48116  ActiveDisplayYMaximum=158.4825
      Scope6 settings: ActiveDisplayYMinimum=408.7005  ActiveDisplayYMaximum=513.4555  DataLoggingVariableName=ScopeData2
      Scope7 settings: ActiveDisplayYMinimum=-5725.99859  ActiveDisplayYMaximum=5883.50444  DataLoggingVariableName=ScopeData3
      Scope8 settings: ActiveDisplayYMinimum=-0.53095  ActiveDisplayYMaximum=4.77853
  Sum : Sum  Inputs=|++
  Switch{,1..3} (4 alike) : Switch  Criteria=u2 > Threshold  SaturateOnIntegerOverflow=off  InputSameDT=off
  Terminator : Terminator
  To Workspace : ToWorkspace  VariableName=batCurrent_A  SampleTime=-1
  To Workspace1 : ToWorkspace  VariableName=Q_inverter  SampleTime=-1
  To Workspace2 : ToWorkspace  VariableName=Q_motor  SampleTime=-1
  To Workspace3 : ToWorkspace  VariableName=Q_charger  SampleTime=-1
  To Workspace4 : ToWorkspace  VariableName=Q_dcdc  SampleTime=-1
  To Workspace5 : ToWorkspace  VariableName=motPwrDemand  SampleTime=-1
  To Workspace6 : ToWorkspace  VariableName=invLoss  SampleTime=-1
  To Workspace7 : ToWorkspace  VariableName=v_veh  SampleTime=-1
  Transfer Fcn{,1..4} (5 alike) : TransferFcn  Denominator=[1 1]
  Unit Delay : UnitDelay  SampleTime=-1
  Unit Delay2 : UnitDelay  SampleTime=-1
  Unit Delay3 : UnitDelay  SampleTime=-1
  UnitDelay : UnitDelay  SampleTime=-1
  I_battery : Outport
  Q_inverter : Outport  Port=2
  Q_motor : Outport  Port=3
  Q_charger : Outport  Port=4
  Q_dcdc : Outport  Port=5
  wires:
  Derivative/1(A) -> Inverter Current vs Acceleration/1, MATLAB Function/2(acceleration_current)
  speed/1 -> Scope12/1, MATLAB Function/1(speed_kph), To Workspace7/1, Inverter Current vs Speed/1, Derivative/1(V)
  Inverter Current vs Speed/1 -> Sum/1
  Inverter Current vs Acceleration/1 -> Sum/2
  Sum/1 -> Saturation/1
  Inverter Heat vs Current/1 -> Transfer Fcn1/1
  Motor Heat vs Current/1 -> Transfer Fcn2/1
  Charger Heat vs Current/1 -> To Workspace3/1, Transfer Fcn3/1
  Transfer Fcn/1 -> Switch/3, Scope15/1
  Transfer Fcn1/1 -> To Workspace1/1, Switch1/3
  Transfer Fcn2/1 -> Scope10/1, To Workspace2/1, Switch3/3
  DCDC Heat vs Current/1 -> Transfer Fcn4/1
  Transfer Fcn4/1 -> Scope16/1, To Workspace4/1, Switch2/3
  Constant2/1 -> MATLAB Function/3(road_grade)
  MATLAB Function/3(lossTq) -> Switch3/1, Gain/1
  Gain/1 -> Scope8/1
  MATLAB Function/4(lossInv) -> Switch1/1, Gain1/1, To Workspace6/1
  Gain1/1 -> Scope13/1
  MATLAB Function/7(Total_power) -> Gain2/1
  Gain2/1 -> Scope2/1
  Constant1/1 -> MATLAB Function/4(U_lo)
  MATLAB Function/8(power_motor_electrical_input) -> To Workspace5/1, Gain3/1
  Constant3/1 -> MATLAB Function/5(U_hi)
  [mfBlower] -> MATLAB Function/6(blowerVF)
  [batTemperature] -> Unit Delay/1
  [SOC] -> Unit Delay2/1
  Gain3/1 -> Scope4/1
  Saturation/1 -> Inverter Heat vs Current/1, Motor Heat vs Current/1, DCDC Heat vs Current/1, Charger Heat vs Current/1, To Workspace/1, Transfer Fcn/1
  MATLAB Function/6(battery_current) -> Switch/1, Scope1/1
  Switch1/1 -> Scope21/1, Q_inverter/1
  Constant4/1 -> Q_charger/1
  Switch2/1 -> Scope23/1, Q_dcdc/1
  MATLAB Function/5(lossDCDC) -> Switch2/1
  Switch3/1 -> Scope22/1, Q_motor/1
  Constant5/1 -> Switch2/2, Switch3/2, Switch1/2, Switch/2
  Switch/1 -> Scope20/1, I_battery/1
  MATLAB Function/1(OCV) -> Scope6/1
  MATLAB Function/2(negSide) -> Scope7/1
  [motPumpPwr] -> UnitDelay/1
  Unit Delay/1 -> Unit Delay3/1, MATLAB Function/9(batTemp)
  UnitDelay/1 -> MATLAB Function/7(motPumpPwr)
  Unit Delay2/1 -> Scope5/1, MATLAB Function/8(SOC)
  Unit Delay3/1 -> MATLAB Function/10(prevBatTemp)
  Transfer Fcn3/1 -> Terminator/1

== system ElectricVehicleThermalManagementWithHeatPump_2026a_version/Battery/Pack 1/Lithium Cell 1RC ==
  note: Power
      | Losses
  C1 : LiBatteryElements_lib/C_table  C_Table=C1_LUT F  SOC_Table=SOC_LUT  Temp_Table=Temperature_LUT K  v0=0 V
  Em_table : LiBatteryElements_lib/Em_table  C_Table=Capacity_LUT hr*A  Em_Table=Em_LUT V  SOC_Table=SOC_LUT  Temp_Table=Temperature_LUT K  Qinit=Qe_init hr*A
  PS-Simulink Converter : nesl_utility/PS-Simulink Converter  PhysicalDomain=network_engine_domain  SubClassName=ps_output  LeftPortType=input  RightPortType=output  PseudoPeriodic=off  Frequencies=[]  VectorFormat=inherit  Unit=inherit  AffineConversion=off
  PS-Simulink Converter1 : nesl_utility/PS-Simulink Converter  PhysicalDomain=network_engine_domain  SubClassName=ps_output  LeftPortType=input  RightPortType=output  PseudoPeriodic=off  Frequencies=[]  VectorFormat=inherit  Unit=inherit  AffineConversion=off
  Power Sum : fl_lib/Physical Signals/Functions/PS Add
  R0 : LiBatteryElements_lib/R_table  R_Table=R0_LUT Ohm  SOC_Table=SOC_LUT  Temp_Table=Temperature_LUT K
  R1 : LiBatteryElements_lib/R_table  R_Table=R1_LUT Ohm  SOC_Table=SOC_LUT  Temp_Table=Temperature_LUT K
  Scope : Scope
      settings: ActiveDisplayYMinimum=0.7814  ActiveDisplayYMaximum=0.94495  DataLoggingVariableName=ScopeData6
  Scope1 : Scope
      settings: ActiveDisplayYMinimum=275.76286  ActiveDisplayYMaximum=280.56079  DataLoggingVariableName=ScopeData7
  To Workspace : ToWorkspace  VariableName=soc_meas  SampleTime=-1
  P : PMIOPort  Side=Left
  + : PMIOPort  Port=2  Side=Left
  T : PMIOPort  Port=3  Side=Right
  - : PMIOPort  Port=4  Side=Right
  tag scope: SOC=global
  wires:
  PS-Simulink Converter/1 -> To Workspace/1, [SOC], Scope/1
  PS-Simulink Converter1/1 -> Scope1/1
  connections:
  R1/RConn2 -- Power Sum/LConn1
  Power Sum/LConn2 -- R0/RConn2
  P/RConn1 -- Power Sum/RConn1
  +/RConn1 -- R0/RConn1
  T/RConn1 -- Em_table/RConn2 -- R0/LConn2 -- C1/LConn2 -- R1/LConn2
  Em_table/LConn1 -- C1/LConn1 -- R1/LConn1
  C1/RConn1 -- R1/RConn1 -- R0/LConn1
  Em_table/RConn1 -- -/RConn1
  C1/LConn3 -- PS-Simulink Converter/LConn1 -- R0/LConn3 -- Em_table/LConn3 -- R1/LConn3
  PS-Simulink Converter1/LConn1 -- Em_table/LConn2

== system ElectricVehicleThermalManagementWithHeatPump_2026a_version/Battery/Pack 1/Thermal Model ==
  Battery Thermal Mass : fl_lib/Thermal/Thermal Elements/Thermal Mass  mass_type=foundation.enum.constant_variable.constant  mass=cell_mass*Ncells kg  sp_heat=cell_Cp_heat J/kg/K  mass_min=1e-6 kg  num_ports=foundation.enum.numPorts2.one  m_specify=off  m_priority=High  m=1 kg  m_nominal_specify=off  m_nominal_value=1  m_nominal_unit=kg  T_specify=on  T_priority=High  T=T_init K  T_nominal_specify=off  T_nominal_value=1  T_nominal_unit=K  Q_specify=off  Q_priority=None  Q=0 W  Q_nominal_specify=off  Q_nominal_value=1  Q_nominal_unit=W
  Controlled Heat Flow Rate Source : fl_lib/Thermal/Thermal Sources/Controlled Heat Flow Rate Source
  Temperature Sensor : fl_lib/Thermal/Thermal Sensors/Temperature Sensor  temperature_measure=foundation.enum.MeasurementReference.difference
  Thermal Reference : fl_lib/Thermal/Thermal Elements/Thermal Reference
  Thermal Reference2 : fl_lib/Thermal/Thermal Elements/Thermal Reference
  H : PMIOPort  Side=Left
  Pxn : PMIOPort  Port=2  Side=Left
  T : PMIOPort  Port=3  Side=Right
  connections:
  H/RConn1 -- Controlled Heat Flow Rate Source/LConn1 -- Battery Thermal Mass/LConn1 -- Temperature Sensor/LConn1
  Pxn/RConn1 -- Controlled Heat Flow Rate Source/RConn1
  Controlled Heat Flow Rate Source/RConn2 -- Thermal Reference2/LConn1
  Thermal Reference/LConn1 -- Temperature Sensor/RConn1
  T/RConn1 -- Temperature Sensor/RConn2

== system ElectricVehicleThermalManagementWithHeatPump_2026a_version/Battery/Pack 2/Lithium Cell 1RC ==
  note: Power
      | Losses
  C1 : LiBatteryElements_lib/C_table  C_Table=C1_LUT F  SOC_Table=SOC_LUT  Temp_Table=Temperature_LUT K  v0=0 V
  Em_table : LiBatteryElements_lib/Em_table  C_Table=Capacity_LUT hr*A  Em_Table=Em_LUT V  SOC_Table=SOC_LUT  Temp_Table=Temperature_LUT K  Qinit=Qe_init hr*A
  Power Sum : fl_lib/Physical Signals/Functions/PS Add
  R0 : LiBatteryElements_lib/R_table  R_Table=R0_LUT Ohm  SOC_Table=SOC_LUT  Temp_Table=Temperature_LUT K
  R1 : LiBatteryElements_lib/R_table  R_Table=R1_LUT Ohm  SOC_Table=SOC_LUT  Temp_Table=Temperature_LUT K
  P : PMIOPort  Side=Left
  + : PMIOPort  Port=2  Side=Left
  T : PMIOPort  Port=3  Side=Right
  - : PMIOPort  Port=4  Side=Right
  connections:
  R1/RConn2 -- Power Sum/LConn1
  Power Sum/LConn2 -- R0/RConn2
  P/RConn1 -- Power Sum/RConn1
  +/RConn1 -- R0/RConn1
  T/RConn1 -- Em_table/RConn2 -- R0/LConn2 -- C1/LConn2 -- R1/LConn2
  Em_table/LConn1 -- C1/LConn1 -- R1/LConn1
  C1/RConn1 -- R1/RConn1 -- R0/LConn1
  Em_table/RConn1 -- -/RConn1
  C1/LConn3 -- Em_table/LConn3 -- R1/LConn3 -- R0/LConn3
